simulink model "tcp_ip"  (R2021b)
settings: Solver=ode5  StartTime=0.0  StopTime=inf  FixedStep=1/20  RelTol=1e-3
PreLoadFcn:
  | mbxruntime.callbacks.PreLoadFcn(bdroot);
PostLoadFcn:
  | mbxruntime.callbacks.PostLoadFcn(bdroot);
InitFcn:
  | mbxruntime.callbacks.InitFcn(bdroot);
StartFcn:
  | mbxruntime.callbacks.StartFcn(bdroot);
StopFcn:
  | mbxruntime.callbacks.StopFcn(bdroot);
model workspace: external: MAT-File .\kea_demo_0218_cs_hws.mat (data not in the file)
undefined symbols (not defined in the file): DiscIntNeverNeededParam, kea_demo_0218_cs_1d5c9b61e8e009e5, kea_demo_0218_cs_4669f259e7287783, kea_demo_0218_cs_87ee11d7829c0052, kea_demo_0218_cs_Audi_A3_1_Dynamics_Simple_initialPitch, kea_demo_0218_cs_Audi_A3_1_Dynamics_Simple_initialRoll, kea_demo_0218_cs_Audi_A3_1_Dynamics_Simple_initialX, kea_demo_0218_cs_Audi_A3_1_Dynamics_Simple_initialY, kea_demo_0218_cs_Audi_A3_1_Dynamics_Simple_initialYaw, kea_demo_0218_cs_Audi_A3_1_Dynamics_Simple_initialZ, kea_demo_0218_cs_Audi_A3_1_PathFollower_Preview_1_PathUniqueID, kea_demo_0218_cs_Roewe_550_S_Sedan_1_Dynamics_Simple_initialX, kea_demo_0218_cs_Roewe_550_S_Sedan_1_Dynamics_Simple_initialY, kea_demo_0218_cs_Roewe_550_S_Sedan_1_Dynamics_Simple_initialYaw, kea_demo_0218_cs_Roewe_550_S_Sedan_1_Dynamics_Simple_initialZ, mbxruntime, warningInitialVelocity, x0
libraries: simulink x56, simulink_extras x18, instrumentlib x2
(part 7 of 7)

== system tcp_ip/Roewe_550_S_Sedan_1/Dynamics_Simple/Chassis/Bicycle_model_[XYZ]/X_Motion/Max RPM and zero- velocity detection ==
  note: Set to zero after infinite small time-step
  note: Zero velocity detection
  ax : Inport
  Drive Torque : Inport  Port=2
  Brake Torque : Inport  Port=3
  v0 : Inport  Port=4
  vx : Inport  Port=5
  Abs : Abs
  Abs1 : Abs
  Compare To Zero : simulink/Logic and Bit Operations/Compare To Zero  relop=<=  OutDataTypeStr=boolean  ZeroCross=off
  Compare To Zero1 : simulink/Logic and Bit Operations/Compare To Zero  relop=>=  OutDataTypeStr=boolean  ZeroCross=off
  Compare To Zero2 : simulink/Logic and Bit Operations/Compare To Zero  relop=>=  OutDataTypeStr=boolean  ZeroCross=off
  Compare To Zero3 : simulink/Logic and Bit Operations/Compare To Zero  relop=<=  OutDataTypeStr=boolean  ZeroCross=off
  Configurable Subsystem : Subsystem  Variant=on  VariantControlMode=label  LabelModeActiveChoice=Continuous
      settings: AttributesFormatString=%<BlockChoice>  OpenFcn=BringToFront(gcb);
  Constant : Constant
  Constant1 : Constant
  Logical Operator : Logic  AllPortsSameDT=off  OutDataTypeStr=boolean
  Logical Operator1 : Logic  AllPortsSameDT=off  OutDataTypeStr=boolean
  Logical Operator2 : Logic  Operator=NOT  AllPortsSameDT=off  OutDataTypeStr=boolean
  Logical Operator3 : Logic  AllPortsSameDT=off  OutDataTypeStr=boolean
  Logical Operator4 : Logic  Operator=OR  AllPortsSameDT=off  OutDataTypeStr=boolean
  Memory : Memory
  Memory1 : Memory
  Memory2 : Memory
  Product : Product  RndMeth=Zero
  Relational Operator : RelationalOperator  Operator=<  OutDataTypeStr=boolean  RndMeth=Nearest
  SR-Memory : Subsystem
  Sum : Sum  Inputs=|-+
  Switch : Switch  Criteria=u2 ~= 0  Threshold=0.5
  ax is 0 : Constant  Value=0
  ax_out : Outport  VectorParamsAs1DForOutWhenUnconnected=off
  vx_reset : Outport  Port=2  VectorParamsAs1DForOutWhenUnconnected=off
  x0 : Outport  Port=3  VectorParamsAs1DForOutWhenUnconnected=off
  wires:
  Logical Operator4/1 -> Logical Operator1/1
  vx/1 -> Compare To Zero/1, Compare To Zero2/1, Memory2/1, Memory/1  "vx"
  Memory2/1 -> Compare To Zero3/1
  Compare To Zero2/1 -> Logical Operator3/1
  Compare To Zero3/1 -> Logical Operator3/2
  Logical Operator3/1 -> Logical Operator4/2  "zero-crossing backward"
  Memory/1 -> Compare To Zero1/1
  Compare To Zero/1 -> Logical Operator/1
  Compare To Zero1/1 -> Logical Operator/2
  Logical Operator/1 -> Logical Operator4/1  "zero-crossing forward"
  Abs/1 -> Relational Operator/1
  Abs1/1 -> Relational Operator/2
  Drive Torque/1 -> Abs/1
  Brake Torque/1 -> Abs1/1
  Relational Operator/1 -> Logical Operator1/2, Logical Operator2/1
  Logical Operator1/1 -> SR-Memory/2(Set)
  Constant/1 -> SR-Memory/1(Signal)
  Logical Operator2/1 -> SR-Memory/3(Reset)
  SR-Memory/1(Out) -> Sum/1, Memory1/1
  Switch/1 -> ax_out/1
  Sum/1 -> Switch/2
  ax is 0/1 -> Switch/3
  Constant1/1 -> Sum/2
  v0/1 -> Product/1
  Product/1 -> x0/1
  Configurable Subsystem/1(Out1) -> Product/2
  ax/1 -> Switch/1  "ax"
  Memory1/1 -> vx_reset/1  "vx"

== system tcp_ip/Roewe_550_S_Sedan_1/Dynamics_Simple/Chassis/Bicycle_model_[XYZ]/Y & Yaw_Motion/Configurable Subsystem ==
  In1 : Inport
  In2 : Inport  Port=2
  Discrete-Time Integrator : Subsystem  VariantControl=Discrete
  Integrator : Subsystem  VariantControl=Continuous
  Out1 : Outport  VectorParamsAs1DForOutWhenUnconnected=off

== system tcp_ip/Roewe_550_S_Sedan_1/Dynamics_Simple/Chassis/Bicycle_model_[XYZ]/Y & Yaw_Motion/Configurable Subsystem1 ==
  In1 : Inport
  Discrete-Time Integrator : Subsystem  VariantControl=Discrete
  Integrator : Subsystem  VariantControl=Continuous
  Out1 : Outport  VectorParamsAs1DForOutWhenUnconnected=off

== system tcp_ip/Roewe_550_S_Sedan_1/Dynamics_Simple/Chassis/Bicycle_model_[XYZ]/Y & Yaw_Motion/Configurable Subsystem2 ==
  In1 : Inport
  In2 : Inport  Port=2
  Discrete-Time Integrator : Subsystem  VariantControl=Discrete
  Integrator : Subsystem  VariantControl=Continuous
  Out1 : Outport  VectorParamsAs1DForOutWhenUnconnected=off

== system tcp_ip/Roewe_550_S_Sedan_1/Dynamics_Simple/Chassis/Bicycle_model_[XYZ]/Z, Pitch_Motion & Roll_Motion/Configurable Subsystem ==
  In1 : Inport
  Discrete-Time Integrator : Subsystem  VariantControl=Discrete
  Integrator : Subsystem  VariantControl=Continuous
  Out1 : Outport  VectorParamsAs1DForOutWhenUnconnected=off

== system tcp_ip/Roewe_550_S_Sedan_1/Dynamics_Simple/Chassis/Bicycle_model_[XYZ]/Z, Pitch_Motion & Roll_Motion/Configurable Subsystem1 ==
  In1 : Inport
  Discrete-Time Integrator : Subsystem  VariantControl=Discrete
  Integrator : Subsystem  VariantControl=Continuous
  Out1 : Outport  VectorParamsAs1DForOutWhenUnconnected=off

== system tcp_ip/Roewe_550_S_Sedan_1/Dynamics_Simple/Chassis/Bicycle_model_[XYZ]/Z, Pitch_Motion & Roll_Motion/Configurable Subsystem2 ==
  In1 : Inport
  Discrete-Time Integrator : Subsystem  VariantControl=Discrete
  Integrator : Subsystem  VariantControl=Continuous
  Out1 : Outport  VectorParamsAs1DForOutWhenUnconnected=off

== system tcp_ip/Roewe_550_S_Sedan_1/Dynamics_Simple/Chassis/Bicycle_model_[XYZ]/Z, Pitch_Motion & Roll_Motion/Configurable Subsystem3 ==
  In1 : Inport
  Discrete-Time Integrator : Subsystem  VariantControl=Discrete
  Integrator : Subsystem  VariantControl=Continuous
  Out1 : Outport  VectorParamsAs1DForOutWhenUnconnected=off

== system tcp_ip/Roewe_550_S_Sedan_1/Dynamics_Simple/Chassis/Bicycle_model_[XYZ]/Z, Pitch_Motion & Roll_Motion/Configurable Subsystem4 ==
  In1 : Inport
  Discrete-Time Integrator : Subsystem  VariantControl=Discrete
  Integrator : Subsystem  VariantControl=Continuous
  Out1 : Outport  VectorParamsAs1DForOutWhenUnconnected=off

== system tcp_ip/Roewe_550_S_Sedan_1/Dynamics_Simple/Chassis/Bicycle_model_[XYZ]/Z, Pitch_Motion & Roll_Motion/Configurable Subsystem5 ==
  In1 : Inport
  Discrete-Time Integrator : Subsystem  VariantControl=Discrete
  Integrator : Subsystem  VariantControl=Continuous
  Out1 : Outport  VectorParamsAs1DForOutWhenUnconnected=off

== system tcp_ip/Roewe_550_S_Sedan_1/Dynamics_Simple/Chassis/Bicycle_model_[XYZ]/Z, Pitch_Motion & Roll_Motion/Configurable Subsystem9 ==
  In1 : Inport
  Derivative : Subsystem  VariantControl=Continuous
  Discrete Derivative : Subsystem  VariantControl=Discrete
      mask Display: dpoly(['k (z-1)'] , ['Ts z'] ,'');
  Out1 : Outport  VectorParamsAs1DForOutWhenUnconnected=off

== system tcp_ip/Roewe_550_S_Sedan_1/Dynamics_Simple/Chassis/FrontTyre/AlphaFront/Enabled Subsystem ==
  In : Inport
  Enable : EnablePort  PropagateVarSize=During execution
  AlphaFront : Fcn  Expr=-atan( (u(2)+u(3)*p.a)/u(1) )
  Alpha : Outport  OutputWhenDisabled=reset  InitialOutput=[0]  VectorParamsAs1DForOutWhenUnconnected=off
  wires:
  AlphaFront/1 -> Alpha/1
  In/1 -> AlphaFront/1

== system tcp_ip/Roewe_550_S_Sedan_1/Dynamics_Simple/Chassis/FrontTyre/Configurable Subsystem/Discrete-Time Integrator ==
  In1 : Inport
  In2 : Inport  Port=2
  Discrete-Time Integrator : DiscreteIntegrator  ExternalReset=level  SampleTime=TimeStep  LimitOutput=on  UpperSaturationLimit=1  LowerSaturationLimit=-1  ICPrevOutput=DiscIntNeverNeededParam  ICPrevScaledInput=DiscIntNeverNeededParam
  Out1 : Outport  VectorParamsAs1DForOutWhenUnconnected=off
  wires:
  Discrete-Time Integrator/1 -> Out1/1
  In2/1 -> Discrete-Time Integrator/2
  In1/1 -> Discrete-Time Integrator/1

== system tcp_ip/Roewe_550_S_Sedan_1/Dynamics_Simple/Chassis/FrontTyre/Configurable Subsystem/Integrator ==
  In1 : Inport
  In2 : Inport  Port=2
  Integrator : Integrator  ExternalReset=level  LimitOutput=on  UpperSaturationLimit=1  LowerSaturationLimit=-1
  Out1 : Outport  VectorParamsAs1DForOutWhenUnconnected=off
  wires:
  Integrator/1 -> Out1/1
  In2/1 -> Integrator/2
  In1/1 -> Integrator/1

== system tcp_ip/Roewe_550_S_Sedan_1/Dynamics_Simple/Chassis/FrontTyre/Configurable Subsystem1/Discrete-Time Integrator ==
  In1 : Inport
  In2 : Inport  Port=2
  Discrete-Time Integrator : DiscreteIntegrator  ExternalReset=level  SampleTime=TimeStep  ICPrevOutput=DiscIntNeverNeededParam  ICPrevScaledInput=DiscIntNeverNeededParam
  Out1 : Outport  VectorParamsAs1DForOutWhenUnconnected=off
  wires:
  Discrete-Time Integrator/1 -> Out1/1
  In2/1 -> Discrete-Time Integrator/2
  In1/1 -> Discrete-Time Integrator/1

== system tcp_ip/Roewe_550_S_Sedan_1/Dynamics_Simple/Chassis/FrontTyre/Configurable Subsystem1/Integrator ==
  In1 : Inport
  In2 : Inport  Port=2
  Integrator : Integrator  ExternalReset=level
  Out1 : Outport  VectorParamsAs1DForOutWhenUnconnected=off
  wires:
  Integrator/1 -> Out1/1
  In2/1 -> Integrator/2
  In1/1 -> Integrator/1

== system tcp_ip/Roewe_550_S_Sedan_1/Dynamics_Simple/Chassis/MuxDynState/Configurable Subsystem1/Discrete-Time Integrator ==
  In1 : Inport
  Discrete-Time Integrator : DiscreteIntegrator  SampleTime=TimeStep  ICPrevOutput=DiscIntNeverNeededParam  ICPrevScaledInput=DiscIntNeverNeededParam
  Out1 : Outport  VectorParamsAs1DForOutWhenUnconnected=off
  wires:
  Discrete-Time Integrator/1 -> Out1/1
  In1/1 -> Discrete-Time Integrator/1

== system tcp_ip/Roewe_550_S_Sedan_1/Dynamics_Simple/Chassis/MuxDynState/Configurable Subsystem1/Integrator ==
  In1 : Inport
  Integrator : Integrator
  Out1 : Outport  VectorParamsAs1DForOutWhenUnconnected=off
  wires:
  Integrator/1 -> Out1/1
  In1/1 -> Integrator/1

== system tcp_ip/Roewe_550_S_Sedan_1/Dynamics_Simple/Chassis/RearTyre/AlphaRear/Enabled Subsystem ==
  In : Inport
  Enable : EnablePort  PropagateVarSize=During execution
  AlphaRear : Fcn  Expr=-atan( (u(2)-u(3)*p.b)/u(1) )
  Alpha : Outport  OutputWhenDisabled=reset  InitialOutput=[0]  VectorParamsAs1DForOutWhenUnconnected=off
  wires:
  AlphaRear/1 -> Alpha/1
  In/1 -> AlphaRear/1

== system tcp_ip/Roewe_550_S_Sedan_1/Dynamics_Simple/Chassis/RearTyre/Configurable Subsystem/Discrete-Time Integrator ==
  In1 : Inport
  In2 : Inport  Port=2
  Discrete-Time Integrator : DiscreteIntegrator  ExternalReset=level  SampleTime=TimeStep  ICPrevOutput=DiscIntNeverNeededParam  ICPrevScaledInput=DiscIntNeverNeededParam
  Out1 : Outport  VectorParamsAs1DForOutWhenUnconnected=off
  wires:
  Discrete-Time Integrator/1 -> Out1/1
  In2/1 -> Discrete-Time Integrator/2
  In1/1 -> Discrete-Time Integrator/1

== system tcp_ip/Roewe_550_S_Sedan_1/Dynamics_Simple/Chassis/RearTyre/Configurable Subsystem/Integrator ==
  In1 : Inport
  In2 : Inport  Port=2
  Integrator : Integrator  ExternalReset=level
  Out1 : Outport  VectorParamsAs1DForOutWhenUnconnected=off
  wires:
  Integrator/1 -> Out1/1
  In2/1 -> Integrator/2
  In1/1 -> Integrator/1

== system tcp_ip/Roewe_550_S_Sedan_1/Dynamics_Simple/Chassis/RearTyre/Configurable Subsystem1/Discrete-Time Integrator ==
  In1 : Inport
  In2 : Inport  Port=2
  Discrete-Time Integrator : DiscreteIntegrator  ExternalReset=level  SampleTime=TimeStep  LimitOutput=on  UpperSaturationLimit=1  LowerSaturationLimit=-1  ICPrevOutput=DiscIntNeverNeededParam  ICPrevScaledInput=DiscIntNeverNeededParam
  Out1 : Outport  VectorParamsAs1DForOutWhenUnconnected=off
  wires:
  Discrete-Time Integrator/1 -> Out1/1
  In2/1 -> Discrete-Time Integrator/2
  In1/1 -> Discrete-Time Integrator/1

== system tcp_ip/Roewe_550_S_Sedan_1/Dynamics_Simple/Chassis/RearTyre/Configurable Subsystem1/Integrator ==
  In1 : Inport
  In2 : Inport  Port=2
  Integrator : Integrator  ExternalReset=level  LimitOutput=on  UpperSaturationLimit=1  LowerSaturationLimit=-1
  Out1 : Outport  VectorParamsAs1DForOutWhenUnconnected=off
  wires:
  Integrator/1 -> Out1/1
  In2/1 -> Integrator/2
  In1/1 -> Integrator/1

== system tcp_ip/Roewe_550_S_Sedan_1/Dynamics_Simple/State2Bus1/state2FullState/limit roll/Substitute 90 & 270 deg (and its plurals) ==
  Angle [rad] : Inport
  270 deg detection : simulink/Model Verification/Check  Static Gap  Description=u <= 269.5 || 270.5 <= u  max=270.5  max_included=on  min=269.5  min_included=on  enabled=on  stopWhenAssertionFail=off  export=on  icon=graphic
      settings: SourceProductBaseCode=SL
  90 deg detection : simulink/Model Verification/Check  Static Gap  Description=u <= 89.5 || 90.5 <= u  max=90.5  max_included=on  min=89.5  min_included=on  enabled=on  stopWhenAssertionFail=off  export=on  icon=graphic
      settings: SourceProductBaseCode=SL
  Angle -360 to +360 deg limiter : Subsystem
  Degrees to Radians : simulink_extras/Transformations/Degrees to Radians
  Radians to Degrees : simulink_extras/Transformations/Radians to Degrees
  Substitution Value : Constant  Value=269.5
  Substitution Value : Constant  Value=89.5
  Switch : Switch  Threshold=0.5
  Switch1 : Switch  Threshold=0.5
  Subst Angle [rad] : Outport  VectorParamsAs1DForOutWhenUnconnected=off
  wires:
  Angle [rad]/1 -> Radians to Degrees/1
  Degrees to Radians/1 -> Subst Angle [rad]/1
  Radians to Degrees/1 -> Angle -360 to +360 deg limiter/1(Angle [deg])
  Switch1/1 -> Degrees to Radians/1
  Substitution Value/1 -> Switch1/3
  270 deg detection/1 -> Switch1/2
  Switch/1 -> Switch1/1, 270 deg detection/1
  Substitution Value/1 -> Switch/3
  90 deg detection/1 -> Switch/2
  Angle -360 to +360 deg limiter/1(LimAngle [deg]) -> 90 deg detection/1, Switch/1

== system tcp_ip/Audi_A3_1/Dynamics_Simple/Chassis/Bicycle_model_[XYZ]/X_Motion/Configurable Subsystem/Discrete-Time Integrator ==
  In1 : Inport
  In2 : Inport  Port=2
  In3 : Inport  Port=3
  Discrete-Time Integrator : DiscreteIntegrator  ExternalReset=level  InitialConditionSource=external  SampleTime=TimeStep  ICPrevOutput=DiscIntNeverNeededParam  ICPrevScaledInput=DiscIntNeverNeededParam
  Out1 : Outport  VectorParamsAs1DForOutWhenUnconnected=off
  wires:
  Discrete-Time Integrator/1 -> Out1/1
  In3/1 -> Discrete-Time Integrator/3
  In2/1 -> Discrete-Time Integrator/2
  In1/1 -> Discrete-Time Integrator/1

== system tcp_ip/Audi_A3_1/Dynamics_Simple/Chassis/Bicycle_model_[XYZ]/X_Motion/Configurable Subsystem/Integrator ==
  In1 : Inport
  In2 : Inport  Port=2
  In3 : Inport  Port=3
  Integrator : Integrator  ExternalReset=level  InitialConditionSource=external
  Out1 : Outport  VectorParamsAs1DForOutWhenUnconnected=off
  wires:
  Integrator/1 -> Out1/1
  In3/1 -> Integrator/3
  In2/1 -> Integrator/2
  In1/1 -> Integrator/1

== system tcp_ip/Audi_A3_1/Dynamics_Simple/Chassis/Bicycle_model_[XYZ]/X_Motion/Configurable Subsystem1/Discrete Torsional damping ==
  In1 : Inport
  Discrete Torsional damping : DiscreteTransferFcn  Numerator="[  1-exp(-( (TimeStep) / 0.1) )  ]"  Denominator="[  1   -exp(-( (TimeStep) / 0.1) )   ]"  SampleTime=TimeStep
  Out1 : Outport  VectorParamsAs1DForOutWhenUnconnected=off
  wires:
  Discrete Torsional damping/1 -> Out1/1
  In1/1 -> Discrete Torsional damping/1

== system tcp_ip/Audi_A3_1/Dynamics_Simple/Chassis/Bicycle_model_[XYZ]/X_Motion/Configurable Subsystem1/Torsional damping ==
  In1 : Inport
  Torsional damping : TransferFcn  Denominator=[0.1 1]
  Out1 : Outport  VectorParamsAs1DForOutWhenUnconnected=off
  wires:
  Torsional damping/1 -> Out1/1
  In1/1 -> Torsional damping/1

== system tcp_ip/Audi_A3_1/Dynamics_Simple/Chassis/Bicycle_model_[XYZ]/X_Motion/Max RPM and zero- velocity detection/Configurable Subsystem ==
  Discrete Step : Subsystem  VariantControl=Discrete
  Step : Subsystem  VariantControl=Continuous
  Out1 : Outport  VectorParamsAs1DForOutWhenUnconnected=off

== system tcp_ip/Audi_A3_1/Dynamics_Simple/Chassis/Bicycle_model_[XYZ]/X_Motion/Max RPM and zero- velocity detection/SR-Memory ==
  Signal : Inport
  Set : Inport  Port=2
  Reset : Inport  Port=3
  Constant : Constant  Value=0
  Detect Rise Positive : simulink/Logic and Bit Operations/Detect Rise Positive  vinit=0  OutDataTypeStr=uint8
  Detect Rise Positive1 : simulink/Logic and Bit Operations/Detect Rise Positive  vinit=0  OutDataTypeStr=uint8
  Manual Switch : ManualSwitch
  Manual Switch1 : ManualSwitch
  Switch : Switch  Criteria=u2 ~= 0
  Switch1 : Switch  Criteria=u2 ~= 0
  Unit Delay : UnitDelay  SampleTime=-1  HasFrameUpgradeWarning=on
  Out : Outport  VectorParamsAs1DForOutWhenUnconnected=off
  wires:
  Constant/1 -> Switch1/1
  Switch/1 -> Switch1/3
  Switch1/1 -> Unit Delay/1, Out/1
  Manual Switch1/1 -> Switch1/2
  Reset/1 -> Manual Switch1/2, Detect Rise Positive1/1
  Detect Rise Positive1/1 -> Manual Switch1/1
  Signal/1 -> Switch/1
  Unit Delay/1 -> Switch/3
  Set/1 -> Detect Rise Positive/1, Manual Switch/2
  Detect Rise Positive/1 -> Manual Switch/1
  Manual Switch/1 -> Switch/2

== system tcp_ip/Audi_A3_1/Dynamics_Simple/Chassis/Bicycle_model_[XYZ]/Y & Yaw_Motion/Configurable Subsystem/Discrete-Time Integrator ==
  In1 : Inport
  In2 : Inport  Port=2
  Discrete-Time Integrator : DiscreteIntegrator  ExternalReset=level  SampleTime=TimeStep  ICPrevOutput=DiscIntNeverNeededParam  ICPrevScaledInput=DiscIntNeverNeededParam
  Out1 : Outport  VectorParamsAs1DForOutWhenUnconnected=off
  wires:
  Discrete-Time Integrator/1 -> Out1/1
  In2/1 -> Discrete-Time Integrator/2
  In1/1 -> Discrete-Time Integrator/1

== system tcp_ip/Audi_A3_1/Dynamics_Simple/Chassis/Bicycle_model_[XYZ]/Y & Yaw_Motion/Configurable Subsystem/Integrator ==
  In1 : Inport
  In2 : Inport  Port=2
  Integrator : Integrator  ExternalReset=level
  Out1 : Outport  VectorParamsAs1DForOutWhenUnconnected=off
  wires:
  Integrator/1 -> Out1/1
  In2/1 -> Integrator/2
  In1/1 -> Integrator/1

== system tcp_ip/Audi_A3_1/Dynamics_Simple/Chassis/Bicycle_model_[XYZ]/Y & Yaw_Motion/Configurable Subsystem1/Discrete-Time Integrator ==
  In1 : Inport
  Discrete-Time Integrator : DiscreteIntegrator  IntegratorMethod=Integration: Backward Euler  SampleTime=TimeStep  ICPrevOutput=DiscIntNeverNeededParam  ICPrevScaledInput=DiscIntNeverNeededParam
  Out1 : Outport  VectorParamsAs1DForOutWhenUnconnected=off
  wires:
  Discrete-Time Integrator/1 -> Out1/1
  In1/1 -> Discrete-Time Integrator/1

== system tcp_ip/Audi_A3_1/Dynamics_Simple/Chassis/Bicycle_model_[XYZ]/Y & Yaw_Motion/Configurable Subsystem1/Integrator ==
  In1 : Inport
  Integrator : Integrator
  Out1 : Outport  VectorParamsAs1DForOutWhenUnconnected=off
  wires:
  Integrator/1 -> Out1/1
  In1/1 -> Integrator/1

== system tcp_ip/Audi_A3_1/Dynamics_Simple/Chassis/Bicycle_model_[XYZ]/Y & Yaw_Motion/Configurable Subsystem2/Discrete-Time Integrator ==
  In1 : Inport
  In2 : Inport  Port=2
  Discrete-Time Integrator : DiscreteIntegrator  ExternalReset=level  SampleTime=TimeStep  ICPrevOutput=DiscIntNeverNeededParam  ICPrevScaledInput=DiscIntNeverNeededParam
  Out1 : Outport  VectorParamsAs1DForOutWhenUnconnected=off
  wires:
  Discrete-Time Integrator/1 -> Out1/1
  In2/1 -> Discrete-Time Integrator/2
  In1/1 -> Discrete-Time Integrator/1

== system tcp_ip/Audi_A3_1/Dynamics_Simple/Chassis/Bicycle_model_[XYZ]/Y & Yaw_Motion/Configurable Subsystem2/Integrator ==
  In1 : Inport
  In2 : Inport  Port=2
  Integrator : Integrator  ExternalReset=level
  Out1 : Outport  VectorParamsAs1DForOutWhenUnconnected=off
  wires:
  Integrator/1 -> Out1/1
  In2/1 -> Integrator/2
  In1/1 -> Integrator/1

== system tcp_ip/Audi_A3_1/Dynamics_Simple/Chassis/Bicycle_model_[XYZ]/Z, Pitch_Motion & Roll_Motion/Configurable Subsystem/Discrete-Time Integrator ==
  In1 : Inport
  Discrete-Time Integrator : DiscreteIntegrator  SampleTime=TimeStep  LimitOutput=on  UpperSaturationLimit=0.087266  LowerSaturationLimit=-0.087266  ICPrevOutput=DiscIntNeverNeededParam  ICPrevScaledInput=DiscIntNeverNeededParam
  Out1 : Outport  VectorParamsAs1DForOutWhenUnconnected=off
  wires:
  Discrete-Time Integrator/1 -> Out1/1
  In1/1 -> Discrete-Time Integrator/1

== system tcp_ip/Audi_A3_1/Dynamics_Simple/Chassis/Bicycle_model_[XYZ]/Z, Pitch_Motion & Roll_Motion/Configurable Subsystem/Integrator ==
  In1 : Inport
  Integrator : Integrator  LimitOutput=on  UpperSaturationLimit=25*pi/180  LowerSaturationLimit=-25*pi/180
  Out1 : Outport  VectorParamsAs1DForOutWhenUnconnected=off
  wires:
  Integrator/1 -> Out1/1
  In1/1 -> Integrator/1

== system tcp_ip/Audi_A3_1/Dynamics_Simple/Chassis/Bicycle_model_[XYZ]/Z, Pitch_Motion & Roll_Motion/Configurable Subsystem1/Discrete-Time Integrator ==
  In1 : Inport
  Discrete-Time Integrator : DiscreteIntegrator  SampleTime=TimeStep  ICPrevOutput=DiscIntNeverNeededParam  ICPrevScaledInput=DiscIntNeverNeededParam
  Out1 : Outport  VectorParamsAs1DForOutWhenUnconnected=off
  wires:
  Discrete-Time Integrator/1 -> Out1/1
  In1/1 -> Discrete-Time Integrator/1

== system tcp_ip/Audi_A3_1/Dynamics_Simple/Chassis/Bicycle_model_[XYZ]/Z, Pitch_Motion & Roll_Motion/Configurable Subsystem1/Integrator ==
  In1 : Inport
  Integrator : Integrator
  Out1 : Outport  VectorParamsAs1DForOutWhenUnconnected=off
  wires:
  Integrator/1 -> Out1/1
  In1/1 -> Integrator/1

== system tcp_ip/Audi_A3_1/Dynamics_Simple/Chassis/Bicycle_model_[XYZ]/Z, Pitch_Motion & Roll_Motion/Configurable Subsystem2/Discrete-Time Integrator ==
  In1 : Inport
  Discrete-Time Integrator : DiscreteIntegrator  SampleTime=TimeStep  ICPrevOutput=DiscIntNeverNeededParam  ICPrevScaledInput=DiscIntNeverNeededParam
  Out1 : Outport  VectorParamsAs1DForOutWhenUnconnected=off
  wires:
  Discrete-Time Integrator/1 -> Out1/1
  In1/1 -> Discrete-Time Integrator/1

== system tcp_ip/Audi_A3_1/Dynamics_Simple/Chassis/Bicycle_model_[XYZ]/Z, Pitch_Motion & Roll_Motion/Configurable Subsystem2/Integrator ==
  In1 : Inport
  Integrator : Integrator
  Out1 : Outport  VectorParamsAs1DForOutWhenUnconnected=off
  wires:
  Integrator/1 -> Out1/1
  In1/1 -> Integrator/1

== system tcp_ip/Audi_A3_1/Dynamics_Simple/Chassis/Bicycle_model_[XYZ]/Z, Pitch_Motion & Roll_Motion/Configurable Subsystem3/Discrete-Time Integrator ==
  In1 : Inport
  Discrete-Time Integrator : DiscreteIntegrator  SampleTime=TimeStep  ICPrevOutput=DiscIntNeverNeededParam  ICPrevScaledInput=DiscIntNeverNeededParam
  Out1 : Outport  VectorParamsAs1DForOutWhenUnconnected=off
  wires:
  Discrete-Time Integrator/1 -> Out1/1
  In1/1 -> Discrete-Time Integrator/1

== system tcp_ip/Audi_A3_1/Dynamics_Simple/Chassis/Bicycle_model_[XYZ]/Z, Pitch_Motion & Roll_Motion/Configurable Subsystem3/Integrator ==
  In1 : Inport
  Integrator : Integrator
  Out1 : Outport  VectorParamsAs1DForOutWhenUnconnected=off
  wires:
  Integrator/1 -> Out1/1
  In1/1 -> Integrator/1

== system tcp_ip/Audi_A3_1/Dynamics_Simple/Chassis/Bicycle_model_[XYZ]/Z, Pitch_Motion & Roll_Motion/Configurable Subsystem4/Discrete-Time Integrator ==
  In1 : Inport
  Discrete-Time Integrator : DiscreteIntegrator  SampleTime=TimeStep  ICPrevOutput=DiscIntNeverNeededParam  ICPrevScaledInput=DiscIntNeverNeededParam
  Out1 : Outport  VectorParamsAs1DForOutWhenUnconnected=off
  wires:
  Discrete-Time Integrator/1 -> Out1/1
  In1/1 -> Discrete-Time Integrator/1

== system tcp_ip/Audi_A3_1/Dynamics_Simple/Chassis/Bicycle_model_[XYZ]/Z, Pitch_Motion & Roll_Motion/Configurable Subsystem4/Integrator ==
  In1 : Inport
  Integrator : Integrator
  Out1 : Outport  VectorParamsAs1DForOutWhenUnconnected=off
  wires:
  Integrator/1 -> Out1/1
  In1/1 -> Integrator/1

== system tcp_ip/Audi_A3_1/Dynamics_Simple/Chassis/Bicycle_model_[XYZ]/Z, Pitch_Motion & Roll_Motion/Configurable Subsystem5/Discrete-Time Integrator ==
  In1 : Inport
  Discrete-Time Integrator : DiscreteIntegrator  SampleTime=TimeStep  ICPrevOutput=DiscIntNeverNeededParam  ICPrevScaledInput=DiscIntNeverNeededParam
  Out1 : Outport  VectorParamsAs1DForOutWhenUnconnected=off
  wires:
  Discrete-Time Integrator/1 -> Out1/1
  In1/1 -> Discrete-Time Integrator/1

== system tcp_ip/Audi_A3_1/Dynamics_Simple/Chassis/Bicycle_model_[XYZ]/Z, Pitch_Motion & Roll_Motion/Configurable Subsystem5/Integrator ==
  In1 : Inport
  Integrator : Integrator
  Out1 : Outport  VectorParamsAs1DForOutWhenUnconnected=off
  wires:
  Integrator/1 -> Out1/1
  In1/1 -> Integrator/1

== system tcp_ip/Audi_A3_1/Dynamics_Simple/Chassis/Bicycle_model_[XYZ]/Z, Pitch_Motion & Roll_Motion/Configurable Subsystem9/Derivative ==
  In1 : Inport
  Derivative : Derivative
  Out1 : Outport  VectorParamsAs1DForOutWhenUnconnected=off
  wires:
  Derivative/1 -> Out1/1
  In1/1 -> Derivative/1

== system tcp_ip/Audi_A3_1/Dynamics_Simple/Chassis/Bicycle_model_[XYZ]/Z, Pitch_Motion & Roll_Motion/Configurable Subsystem9/Discrete Derivative ==
  In1 : Inport
  Discrete Derivative : simulink/Discrete/Discrete Derivative  gainval=1.0  ICPrevScaledInput=0.0  OutMin=[]  OutMax=[]  OutDataType=fixdt(1, 16)  OutScaling=2^-10  DoSatur=off
  Out1 : Outport  VectorParamsAs1DForOutWhenUnconnected=off
  wires:
  Discrete Derivative/1 -> Out1/1
  In1/1 -> Discrete Derivative/1

== system tcp_ip/Audi_A3_1/Dynamics_Simple/State2Bus1/state2FullState/limit roll/Substitute 90 & 270 deg (and its plurals)/Angle -360 to +360 deg limiter ==
  Angle [deg] : Inport
  Constant : Constant  Value=360
  Gain : Gain  Gain=1/720
  Gain1 : Gain  Gain=720
  Rounding Function : Rounding
  Sum : Sum  Inputs=|-+
  Sum1 : Sum  Inputs=|++
  LimAngle [deg] : Outport  VectorParamsAs1DForOutWhenUnconnected=off
  wires:
  Constant/1 -> Sum1/2
  Sum1/1 -> Gain/1
  Angle [deg]/1 -> Sum/2, Sum1/1
  Gain/1 -> Rounding Function/1
  Rounding Function/1 -> Gain1/1
  Gain1/1 -> Sum/1
  Sum/1 -> LimAngle [deg]/1

== system tcp_ip/Roewe_550_S_Sedan_1/Dynamics_Simple/Chassis/Bicycle_model_[XYZ]/X_Motion/Configurable Subsystem/Discrete-Time Integrator ==
  In1 : Inport
  In2 : Inport  Port=2
  In3 : Inport  Port=3
  Discrete-Time Integrator : DiscreteIntegrator  ExternalReset=level  InitialConditionSource=external  SampleTime=TimeStep  ICPrevOutput=DiscIntNeverNeededParam  ICPrevScaledInput=DiscIntNeverNeededParam
  Out1 : Outport  VectorParamsAs1DForOutWhenUnconnected=off
  wires:
  Discrete-Time Integrator/1 -> Out1/1
  In3/1 -> Discrete-Time Integrator/3
  In2/1 -> Discrete-Time Integrator/2
  In1/1 -> Discrete-Time Integrator/1

== system tcp_ip/Roewe_550_S_Sedan_1/Dynamics_Simple/Chassis/Bicycle_model_[XYZ]/X_Motion/Configurable Subsystem/Integrator ==
  In1 : Inport
  In2 : Inport  Port=2
  In3 : Inport  Port=3
  Integrator : Integrator  ExternalReset=level  InitialConditionSource=external
  Out1 : Outport  VectorParamsAs1DForOutWhenUnconnected=off
  wires:
  Integrator/1 -> Out1/1
  In3/1 -> Integrator/3
  In2/1 -> Integrator/2
  In1/1 -> Integrator/1

== system tcp_ip/Roewe_550_S_Sedan_1/Dynamics_Simple/Chassis/Bicycle_model_[XYZ]/X_Motion/Configurable Subsystem1/Discrete Torsional damping ==
  In1 : Inport
  Discrete Torsional damping : DiscreteTransferFcn  Numerator="[  1-exp(-( (TimeStep) / 0.1) )  ]"  Denominator="[  1   -exp(-( (TimeStep) / 0.1) )   ]"  SampleTime=TimeStep
  Out1 : Outport  VectorParamsAs1DForOutWhenUnconnected=off
  wires:
  Discrete Torsional damping/1 -> Out1/1
  In1/1 -> Discrete Torsional damping/1

== system tcp_ip/Roewe_550_S_Sedan_1/Dynamics_Simple/Chassis/Bicycle_model_[XYZ]/X_Motion/Configurable Subsystem1/Torsional damping ==
  In1 : Inport
  Torsional damping : TransferFcn  Denominator=[0.1 1]
  Out1 : Outport  VectorParamsAs1DForOutWhenUnconnected=off
  wires:
  Torsional damping/1 -> Out1/1
  In1/1 -> Torsional damping/1

== system tcp_ip/Roewe_550_S_Sedan_1/Dynamics_Simple/Chassis/Bicycle_model_[XYZ]/X_Motion/Max RPM and zero- velocity detection/Configurable Subsystem ==
  Discrete Step : Subsystem  VariantControl=Discrete
  Step : Subsystem  VariantControl=Continuous
  Out1 : Outport  VectorParamsAs1DForOutWhenUnconnected=off

== system tcp_ip/Roewe_550_S_Sedan_1/Dynamics_Simple/Chassis/Bicycle_model_[XYZ]/X_Motion/Max RPM and zero- velocity detection/SR-Memory ==
  Signal : Inport
  Set : Inport  Port=2
  Reset : Inport  Port=3
  Constant : Constant  Value=0
  Detect Rise Positive : simulink/Logic and Bit Operations/Detect Rise Positive  vinit=0  OutDataTypeStr=uint8
  Detect Rise Positive1 : simulink/Logic and Bit Operations/Detect Rise Positive  vinit=0  OutDataTypeStr=uint8
  Manual Switch : ManualSwitch
  Manual Switch1 : ManualSwitch
  Switch : Switch  Criteria=u2 ~= 0
  Switch1 : Switch  Criteria=u2 ~= 0
  Unit Delay : UnitDelay  SampleTime=-1  HasFrameUpgradeWarning=on
  Out : Outport  VectorParamsAs1DForOutWhenUnconnected=off
  wires:
  Constant/1 -> Switch1/1
  Switch/1 -> Switch1/3
  Switch1/1 -> Unit Delay/1, Out/1
  Manual Switch1/1 -> Switch1/2
  Reset/1 -> Manual Switch1/2, Detect Rise Positive1/1
  Detect Rise Positive1/1 -> Manual Switch1/1
  Signal/1 -> Switch/1
  Unit Delay/1 -> Switch/3
  Set/1 -> Detect Rise Positive/1, Manual Switch/2
  Detect Rise Positive/1 -> Manual Switch/1
  Manual Switch/1 -> Switch/2

== system tcp_ip/Roewe_550_S_Sedan_1/Dynamics_Simple/Chassis/Bicycle_model_[XYZ]/Y & Yaw_Motion/Configurable Subsystem/Discrete-Time Integrator ==
  In1 : Inport
  In2 : Inport  Port=2
  Discrete-Time Integrator : DiscreteIntegrator  ExternalReset=level  SampleTime=TimeStep  ICPrevOutput=DiscIntNeverNeededParam  ICPrevScaledInput=DiscIntNeverNeededParam
  Out1 : Outport  VectorParamsAs1DForOutWhenUnconnected=off
  wires:
  Discrete-Time Integrator/1 -> Out1/1
  In2/1 -> Discrete-Time Integrator/2
  In1/1 -> Discrete-Time Integrator/1

== system tcp_ip/Roewe_550_S_Sedan_1/Dynamics_Simple/Chassis/Bicycle_model_[XYZ]/Y & Yaw_Motion/Configurable Subsystem/Integrator ==
  In1 : Inport
  In2 : Inport  Port=2
  Integrator : Integrator  ExternalReset=level
  Out1 : Outport  VectorParamsAs1DForOutWhenUnconnected=off
  wires:
  Integrator/1 -> Out1/1
  In2/1 -> Integrator/2
  In1/1 -> Integrator/1

== system tcp_ip/Roewe_550_S_Sedan_1/Dynamics_Simple/Chassis/Bicycle_model_[XYZ]/Y & Yaw_Motion/Configurable Subsystem1/Discrete-Time Integrator ==
  In1 : Inport
  Discrete-Time Integrator : DiscreteIntegrator  IntegratorMethod=Integration: Backward Euler  SampleTime=TimeStep  ICPrevOutput=DiscIntNeverNeededParam  ICPrevScaledInput=DiscIntNeverNeededParam
  Out1 : Outport  VectorParamsAs1DForOutWhenUnconnected=off
  wires:
  Discrete-Time Integrator/1 -> Out1/1
  In1/1 -> Discrete-Time Integrator/1

== system tcp_ip/Roewe_550_S_Sedan_1/Dynamics_Simple/Chassis/Bicycle_model_[XYZ]/Y & Yaw_Motion/Configurable Subsystem1/Integrator ==
  In1 : Inport
  Integrator : Integrator
  Out1 : Outport  VectorParamsAs1DForOutWhenUnconnected=off
  wires:
  Integrator/1 -> Out1/1
  In1/1 -> Integrator/1

== system tcp_ip/Roewe_550_S_Sedan_1/Dynamics_Simple/Chassis/Bicycle_model_[XYZ]/Y & Yaw_Motion/Configurable Subsystem2/Discrete-Time Integrator ==
  In1 : Inport
  In2 : Inport  Port=2
  Discrete-Time Integrator : DiscreteIntegrator  ExternalReset=level  SampleTime=TimeStep  ICPrevOutput=DiscIntNeverNeededParam  ICPrevScaledInput=DiscIntNeverNeededParam
  Out1 : Outport  VectorParamsAs1DForOutWhenUnconnected=off
  wires:
  Discrete-Time Integrator/1 -> Out1/1
  In2/1 -> Discrete-Time Integrator/2
  In1/1 -> Discrete-Time Integrator/1

== system tcp_ip/Roewe_550_S_Sedan_1/Dynamics_Simple/Chassis/Bicycle_model_[XYZ]/Y & Yaw_Motion/Configurable Subsystem2/Integrator ==
  In1 : Inport
  In2 : Inport  Port=2
  Integrator : Integrator  ExternalReset=level
  Out1 : Outport  VectorParamsAs1DForOutWhenUnconnected=off
  wires:
  Integrator/1 -> Out1/1
  In2/1 -> Integrator/2
  In1/1 -> Integrator/1

== system tcp_ip/Roewe_550_S_Sedan_1/Dynamics_Simple/Chassis/Bicycle_model_[XYZ]/Z, Pitch_Motion & Roll_Motion/Configurable Subsystem/Discrete-Time Integrator ==
  In1 : Inport
  Discrete-Time Integrator : DiscreteIntegrator  SampleTime=TimeStep  LimitOutput=on  UpperSaturationLimit=0.087266  LowerSaturationLimit=-0.087266  ICPrevOutput=DiscIntNeverNeededParam  ICPrevScaledInput=DiscIntNeverNeededParam
  Out1 : Outport  VectorParamsAs1DForOutWhenUnconnected=off
  wires:
  Discrete-Time Integrator/1 -> Out1/1
  In1/1 -> Discrete-Time Integrator/1

== system tcp_ip/Roewe_550_S_Sedan_1/Dynamics_Simple/Chassis/Bicycle_model_[XYZ]/Z, Pitch_Motion & Roll_Motion/Configurable Subsystem/Integrator ==
  In1 : Inport
  Integrator : Integrator  LimitOutput=on  UpperSaturationLimit=25*pi/180  LowerSaturationLimit=-25*pi/180
  Out1 : Outport  VectorParamsAs1DForOutWhenUnconnected=off
  wires:
  Integrator/1 -> Out1/1
  In1/1 -> Integrator/1

== system tcp_ip/Roewe_550_S_Sedan_1/Dynamics_Simple/Chassis/Bicycle_model_[XYZ]/Z, Pitch_Motion & Roll_Motion/Configurable Subsystem1/Discrete-Time Integrator ==
  In1 : Inport
  Discrete-Time Integrator : DiscreteIntegrator  SampleTime=TimeStep  ICPrevOutput=DiscIntNeverNeededParam  ICPrevScaledInput=DiscIntNeverNeededParam
  Out1 : Outport  VectorParamsAs1DForOutWhenUnconnected=off
  wires:
  Discrete-Time Integrator/1 -> Out1/1
  In1/1 -> Discrete-Time Integrator/1

== system tcp_ip/Roewe_550_S_Sedan_1/Dynamics_Simple/Chassis/Bicycle_model_[XYZ]/Z, Pitch_Motion & Roll_Motion/Configurable Subsystem1/Integrator ==
  In1 : Inport
  Integrator : Integrator
  Out1 : Outport  VectorParamsAs1DForOutWhenUnconnected=off
  wires:
  Integrator/1 -> Out1/1
  In1/1 -> Integrator/1

== system tcp_ip/Roewe_550_S_Sedan_1/Dynamics_Simple/Chassis/Bicycle_model_[XYZ]/Z, Pitch_Motion & Roll_Motion/Configurable Subsystem2/Discrete-Time Integrator ==
  In1 : Inport
  Discrete-Time Integrator : DiscreteIntegrator  SampleTime=TimeStep  ICPrevOutput=DiscIntNeverNeededParam  ICPrevScaledInput=DiscIntNeverNeededParam
  Out1 : Outport  VectorParamsAs1DForOutWhenUnconnected=off
  wires:
  Discrete-Time Integrator/1 -> Out1/1
  In1/1 -> Discrete-Time Integrator/1

== system tcp_ip/Roewe_550_S_Sedan_1/Dynamics_Simple/Chassis/Bicycle_model_[XYZ]/Z, Pitch_Motion & Roll_Motion/Configurable Subsystem2/Integrator ==
  In1 : Inport
  Integrator : Integrator
  Out1 : Outport  VectorParamsAs1DForOutWhenUnconnected=off
  wires:
  Integrator/1 -> Out1/1
  In1/1 -> Integrator/1

== system tcp_ip/Roewe_550_S_Sedan_1/Dynamics_Simple/Chassis/Bicycle_model_[XYZ]/Z, Pitch_Motion & Roll_Motion/Configurable Subsystem3/Discrete-Time Integrator ==
  In1 : Inport
  Discrete-Time Integrator : DiscreteIntegrator  SampleTime=TimeStep  ICPrevOutput=DiscIntNeverNeededParam  ICPrevScaledInput=DiscIntNeverNeededParam
  Out1 : Outport  VectorParamsAs1DForOutWhenUnconnected=off
  wires:
  Discrete-Time Integrator/1 -> Out1/1
  In1/1 -> Discrete-Time Integrator/1

== system tcp_ip/Roewe_550_S_Sedan_1/Dynamics_Simple/Chassis/Bicycle_model_[XYZ]/Z, Pitch_Motion & Roll_Motion/Configurable Subsystem3/Integrator ==
  In1 : Inport
  Integrator : Integrator
  Out1 : Outport  VectorParamsAs1DForOutWhenUnconnected=off
  wires:
  Integrator/1 -> Out1/1
  In1/1 -> Integrator/1

== system tcp_ip/Roewe_550_S_Sedan_1/Dynamics_Simple/Chassis/Bicycle_model_[XYZ]/Z, Pitch_Motion & Roll_Motion/Configurable Subsystem4/Discrete-Time Integrator ==
  In1 : Inport
  Discrete-Time Integrator : DiscreteIntegrator  SampleTime=TimeStep  ICPrevOutput=DiscIntNeverNeededParam  ICPrevScaledInput=DiscIntNeverNeededParam
  Out1 : Outport  VectorParamsAs1DForOutWhenUnconnected=off
  wires:
  Discrete-Time Integrator/1 -> Out1/1
  In1/1 -> Discrete-Time Integrator/1

== system tcp_ip/Roewe_550_S_Sedan_1/Dynamics_Simple/Chassis/Bicycle_model_[XYZ]/Z, Pitch_Motion & Roll_Motion/Configurable Subsystem4/Integrator ==
  In1 : Inport
  Integrator : Integrator
  Out1 : Outport  VectorParamsAs1DForOutWhenUnconnected=off
  wires:
  Integrator/1 -> Out1/1
  In1/1 -> Integrator/1

== system tcp_ip/Roewe_550_S_Sedan_1/Dynamics_Simple/Chassis/Bicycle_model_[XYZ]/Z, Pitch_Motion & Roll_Motion/Configurable Subsystem5/Discrete-Time Integrator ==
  In1 : Inport
  Discrete-Time Integrator : DiscreteIntegrator  SampleTime=TimeStep  ICPrevOutput=DiscIntNeverNeededParam  ICPrevScaledInput=DiscIntNeverNeededParam
  Out1 : Outport  VectorParamsAs1DForOutWhenUnconnected=off
  wires:
  Discrete-Time Integrator/1 -> Out1/1
  In1/1 -> Discrete-Time Integrator/1

== system tcp_ip/Roewe_550_S_Sedan_1/Dynamics_Simple/Chassis/Bicycle_model_[XYZ]/Z, Pitch_Motion & Roll_Motion/Configurable Subsystem5/Integrator ==
  In1 : Inport
  Integrator : Integrator
  Out1 : Outport  VectorParamsAs1DForOutWhenUnconnected=off
  wires:
  Integrator/1 -> Out1/1
  In1/1 -> Integrator/1

== system tcp_ip/Roewe_550_S_Sedan_1/Dynamics_Simple/Chassis/Bicycle_model_[XYZ]/Z, Pitch_Motion & Roll_Motion/Configurable Subsystem9/Derivative ==
  In1 : Inport
  Derivative : Derivative
  Out1 : Outport  VectorParamsAs1DForOutWhenUnconnected=off
  wires:
  Derivative/1 -> Out1/1
  In1/1 -> Derivative/1

== system tcp_ip/Roewe_550_S_Sedan_1/Dynamics_Simple/Chassis/Bicycle_model_[XYZ]/Z, Pitch_Motion & Roll_Motion/Configurable Subsystem9/Discrete Derivative ==
  In1 : Inport
  Discrete Derivative : simulink/Discrete/Discrete Derivative  gainval=1.0  ICPrevScaledInput=0.0  OutMin=[]  OutMax=[]  OutDataType=fixdt(1, 16)  OutScaling=2^-10  DoSatur=off
  Out1 : Outport  VectorParamsAs1DForOutWhenUnconnected=off
  wires:
  Discrete Derivative/1 -> Out1/1
  In1/1 -> Discrete Derivative/1

== system tcp_ip/Roewe_550_S_Sedan_1/Dynamics_Simple/State2Bus1/state2FullState/limit roll/Substitute 90 & 270 deg (and its plurals)/Angle -360 to +360 deg limiter ==
  Angle [deg] : Inport
  Constant : Constant  Value=360
  Gain : Gain  Gain=1/720
  Gain1 : Gain  Gain=720
  Rounding Function : Rounding
  Sum : Sum  Inputs=|-+
  Sum1 : Sum  Inputs=|++
  LimAngle [deg] : Outport  VectorParamsAs1DForOutWhenUnconnected=off
  wires:
  Constant/1 -> Sum1/2
  Sum1/1 -> Gain/1
  Angle [deg]/1 -> Sum/2, Sum1/1
  Gain/1 -> Rounding Function/1
  Rounding Function/1 -> Gain1/1
  Gain1/1 -> Sum/1
  Sum/1 -> LimAngle [deg]/1

== system tcp_ip/Audi_A3_1/Dynamics_Simple/Chassis/Bicycle_model_[XYZ]/X_Motion/Max RPM and zero- velocity detection/Configurable Subsystem/Discrete Step ==
  Discrete Step : Step  Time=0.0001  Before=1  After=0  SampleTime=TimeStep
  Out1 : Outport  VectorParamsAs1DForOutWhenUnconnected=off
  wires:
  Discrete Step/1 -> Out1/1

== system tcp_ip/Audi_A3_1/Dynamics_Simple/Chassis/Bicycle_model_[XYZ]/X_Motion/Max RPM and zero- velocity detection/Configurable Subsystem/Step ==
  Step : Step  Time=0.0001  Before=1  After=0  SampleTime=0
  Out1 : Outport  VectorParamsAs1DForOutWhenUnconnected=off
  wires:
  Step/1 -> Out1/1

== system tcp_ip/Roewe_550_S_Sedan_1/Dynamics_Simple/Chassis/Bicycle_model_[XYZ]/X_Motion/Max RPM and zero- velocity detection/Configurable Subsystem/Discrete Step ==
  Discrete Step : Step  Time=0.0001  Before=1  After=0  SampleTime=TimeStep
  Out1 : Outport  VectorParamsAs1DForOutWhenUnconnected=off
  wires:
  Discrete Step/1 -> Out1/1

== system tcp_ip/Roewe_550_S_Sedan_1/Dynamics_Simple/Chassis/Bicycle_model_[XYZ]/X_Motion/Max RPM and zero- velocity detection/Configurable Subsystem/Step ==
  Step : Step  Time=0.0001  Before=1  After=0  SampleTime=0
  Out1 : Outport  VectorParamsAs1DForOutWhenUnconnected=off
  wires:
  Step/1 -> Out1/1

== matlab function tcp_ip/Roewe_550_S_Sedan_1/PathFollower_Preview_1/LateralController/Calculate delta wheel/eml_delta_steering_error ==
  data: v_x_vehicle input; v_x_vehicle_Min input; t_Preview_LatCtrl input; delta_steeringwheeltotal output; v_y_vehicle input; yawrate_vehicle input; CorneringStiffness_Tyres_Front input; CorneringStiffness_Tyres_Rear input; m_vehicle_total input; inertia_z_vehicle_total input; e_Lat input size=10; Pos_x_CoG_Vehicle input; wheelbase input; RefreshCounter parameter
function delta_steeringwheeltotal = eml_delta_steering_error(v_x_vehicle,v_x_vehicle_Min,t_Preview_LatCtrl,v_y_vehicle,yawrate_vehicle,CorneringStiffness_Tyres_Front,CorneringStiffness_Tyres_Rear,m_vehicle_total,inertia_z_vehicle_total,e_Lat,Pos_x_CoG_Vehicle,wheelbase,RefreshCounter)

delta_steeringwheeltotal = emlfcn_delta_steering_error(v_x_vehicle,v_x_vehicle_Min,t_Preview_LatCtrl,v_y_vehicle,yawrate_vehicle,CorneringStiffness_Tyres_Front,CorneringStiffness_Tyres_Rear,m_vehicle_total,inertia_z_vehicle_total,e_Lat,Pos_x_CoG_Vehicle,wheelbase,RefreshCounter);

% end function

== matlab function tcp_ip/Roewe_550_S_Sedan_1/MATLAB Function ==
  data: x input; y output

    function y = calculateY(x)
    if x > 50
        y = 5;
    elseif x > 30
        y = 10;
    elseif x > 10
        y = 14;
    else
        y = 20;
    end
end

== matlab function tcp_ip/Audi_A3_1/PathFollower_Preview_1/LateralController/Calculate delta wheel/eml_delta_steering_error ==
  data: v_x_vehicle input; v_x_vehicle_Min input; t_Preview_LatCtrl input; delta_steeringwheeltotal output; v_y_vehicle input; yawrate_vehicle input; CorneringStiffness_Tyres_Front input; CorneringStiffness_Tyres_Rear input; m_vehicle_total input; inertia_z_vehicle_total input; e_Lat input size=10; Pos_x_CoG_Vehicle input; wheelbase input; RefreshCounter parameter
function delta_steeringwheeltotal = eml_delta_steering_error(v_x_vehicle,v_x_vehicle_Min,t_Preview_LatCtrl,v_y_vehicle,yawrate_vehicle,CorneringStiffness_Tyres_Front,CorneringStiffness_Tyres_Rear,m_vehicle_total,inertia_z_vehicle_total,e_Lat,Pos_x_CoG_Vehicle,wheelbase,RefreshCounter)

delta_steeringwheeltotal = emlfcn_delta_steering_error(v_x_vehicle,v_x_vehicle_Min,t_Preview_LatCtrl,v_y_vehicle,yawrate_vehicle,CorneringStiffness_Tyres_Front,CorneringStiffness_Tyres_Rear,m_vehicle_total,inertia_z_vehicle_total,e_Lat,Pos_x_CoG_Vehicle,wheelbase,RefreshCounter);

% end function
